simulink model "exemplefir"  (Simulink 7.1)
settings: Solver=FixedStepDiscrete  StartTime=0.0  StopTime=10.0  FixedStep=0.001  RelTol=1e-3
undefined symbols (not defined in the file or in its folder): get, magnitude
libraries: dspbuff3 x2, dspxfrm3 x2, dspsnks4 x2, dspsrcs4 x2, dspsigops x2
settings Model: Creator=Administrateur  LastModifiedBy=Administrateur
settings OptimizationCC: OptimizeModelRefInitCode=on  LifeSpan=1
settings HardwareCC: ProdBitPerInt=16  ProdEndianess=LittleEndian  ProdWordSize=16  ProdHWDeviceType=16-bit Generic
settings RTWCC: SystemTargetFile=dspic.tlc  TemplateMakefile=dspic_pic30_gcc.tmf  PostCodeGenCommand=dsPIC_Compile()  Description=Embedded Target for Microchip dsPIC (real-time)  ProcessScript=dspic_make_rtw_hook
settings CodeAppCC: IgnoreCustomStorageClasses=off
settings STFCustomTargetCC: ModelReferenceCompliant=off  IncludeMdlTerminateFcn=off  CombineOutputUpdateFcns=on  SuppressErrorStatus=on  ERTCustomFileBanners=on  SupportContinuousTime=off  SupportNonInlinedSFcns=off  SystemTargetFile=dspic.tlc
settings ERTTargetCC: ModelReferenceCompliant=off  CompOptLevelCompliant=off  IncludeMdlTerminateFcn=off  SuppressErrorStatus=on  ERTFirstTimeCompliant=off  ModelStepFunctionPrototypeControlCompliant=off  ExtModeMexFile=noextcomm  InlinedParameterPlacement=NonHierarchical  ERTSrcFileBannerTemplate=dsPIC_code_template.cgt  ERTHdrFileBannerTemplate=dsPIC_code_template.cgt  ERTDataSrcFileTemplate=dsPIC_code_template.cgt  ERTDataHdrFileTemplate=dsPIC_code_template.cgt  ERTCustomFileTemplate=dsPIC_main.tlc
settings CustomProperty: DataType=string  Value=C:\PROGRA~1\MATLAB\R2008a\bin\win32\gmake

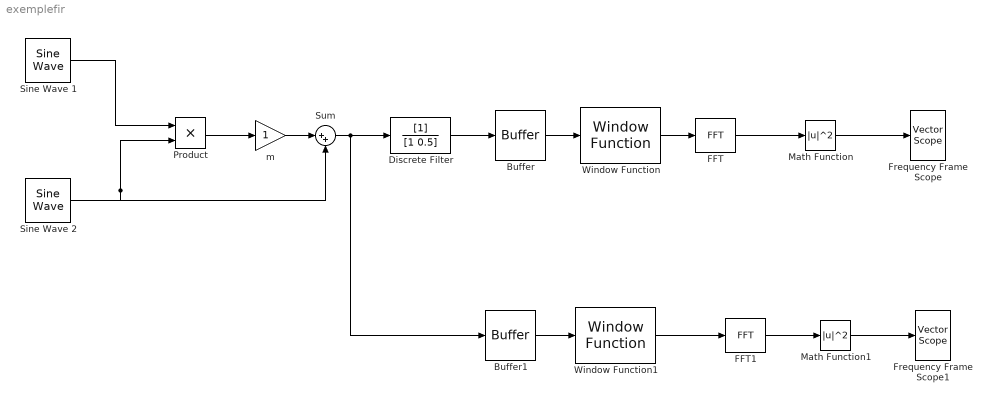
== system exemplefir ==
  Buffer : dspbuff3/Buffer  N=64  V=0  ic=0
  Buffer1 : dspbuff3/Buffer  N=64  V=0  ic=0
  Discrete Filter : DiscreteFilter  Denominator=[1 0.5]  SampleTime=0.1
  FFT : dspxfrm3/FFT  DialogController=dspDDGCreate  DialogControllerArgs=DataTag0  CompMethod=Table lookup  TableOpt=Speed  BitRevOrder=off  InheritFFTLength=on  FFTLength=64  SkipNorm=on  roundingMode=Floor  overflowMode=off
  FFT1 : dspxfrm3/FFT  DialogController=dspDDGCreate  DialogControllerArgs=DataTag1  CompMethod=Table lookup  TableOpt=Speed  BitRevOrder=off  InheritFFTLength=on  FFTLength=64  SkipNorm=on  roundingMode=Floor  overflowMode=off
  Frequency Frame Scope : dspsnks4/Vector Scope  DialogController=dspdialog.VectorScope  DialogControllerArgs=DataTag2  ScopeProperties=on  Domain=Frequency  HorizSpan=1  DisplayProperties=off  AxisGrid=on  Memory=off  FrameNumber=on  AxisLegend=off  AxisZoom=off  OpenScopeAtSimStart=on  OpenScopeImmediately=off  FigPos=get(0,'defaultfigureposition')  AxisProperties=off  XUnits=Hertz  XRange=[0...Fs/2]  InheritXIncr=on  XIncr=1  XLabel=Time  XLimit=Auto  XMin=0  XMax=1  XStart=0  YUnits=dB  YLabel=Amplitude  LineProperties=off
      settings: YMin=-10  YMax=10
  Frequency Frame Scope1 : dspsnks4/Vector Scope  DialogController=dspdialog.VectorScope  DialogControllerArgs=DataTag3  ScopeProperties=on  Domain=Frequency  HorizSpan=1  DisplayProperties=off  AxisGrid=on  Memory=off  FrameNumber=on  AxisLegend=off  AxisZoom=off  OpenScopeAtSimStart=on  OpenScopeImmediately=off  FigPos=get(0,'defaultfigureposition')  AxisProperties=off  XUnits=Hertz  XRange=[0...Fs/2]  InheritXIncr=on  XIncr=1  XLabel=Time  XLimit=Auto  XMin=0  XMax=1  XStart=0  YUnits=dB  YLabel=Amplitude  LineProperties=off
      settings: YMin=-10  YMax=10
  Math Function : Math  Operator=magnitude^2  OutDataType=sfix(16)  OutScaling=2^0  SaturateOnIntegerOverflow=on
  Math Function1 : Math  Operator=magnitude^2  OutDataType=sfix(16)  OutScaling=2^0  SaturateOnIntegerOverflow=on
  Product : Product  OutDataType=sfix(16)  OutScaling=2^0  RndMeth=Zero
  Sine Wave 1 : dspsrcs4/Sine Wave  Amplitude=1  Frequency=100  Phase=0  SampleMode=Discrete  OutComplex=Real  CompMethod=Trigonometric fcn  TableSize=Speed  SampleTime=1/10  SamplesPerFrame=1  dataType=double  wordLen=16  udDataType=sfix(16)  fracBitsMode=Best precision  numFracBits=15  ResetState=Restart at time zero
  Sine Wave 2 : dspsrcs4/Sine Wave  Amplitude=1  Frequency=100  Phase=0  SampleMode=Discrete  OutComplex=Real  CompMethod=Trigonometric fcn  TableSize=Speed  SampleTime=1/10  SamplesPerFrame=1  dataType=double  wordLen=16  udDataType=sfix(16)  fracBitsMode=Best precision  numFracBits=15  ResetState=Restart at time zero
  Sum : Sum  Inputs=|++  OutDataType=sfix(16)  OutScaling=2^0
  Window Function : dspsigops/Window Function  DialogController=dspDDGCreate  DialogControllerArgs=DataTag4  winmode=Apply window to input  wintype=Boxcar  sampmode=Continuous  samptime=1  N=64  Rs=50  beta=10  winsamp=Symmetric  UserWindow=hamming  OptParams=off  UserParams={'symmetric'}  dataType=double  isSigned=on  wordLen=16  udDataType=sfix(16)  fracBitsMode=Best precision  numFracBits=15  roundingMode=Floor  overflowMode=off  numSidelobes=4  sidelobeLevel=-30
  Window Function1 : dspsigops/Window Function  DialogController=dspDDGCreate  DialogControllerArgs=DataTag5  winmode=Apply window to input  wintype=Boxcar  sampmode=Continuous  samptime=1  N=64  Rs=50  beta=10  winsamp=Symmetric  UserWindow=hamming  OptParams=off  UserParams={'symmetric'}  dataType=double  isSigned=on  wordLen=16  udDataType=sfix(16)  fracBitsMode=Best precision  numFracBits=15  roundingMode=Floor  overflowMode=off  numSidelobes=4  sidelobeLevel=-30
  m : Gain  ParameterDataType=sfix(16)  ParameterScaling=2^0  OutDataType=sfix(16)  OutScaling=2^0
  wires:
  Sine Wave 1/1 -> Product/1
  Sine Wave 2/1 -> Product/2, Sum/2
  Product/1 -> m/1
  m/1 -> Sum/1
  Discrete Filter/1 -> Buffer/1
  FFT/1 -> Math Function/1
  Buffer/1 -> Window Function/1
  Window Function/1 -> FFT/1
  Math Function/1 -> Frequency Frame Scope/1
  FFT1/1 -> Math Function1/1
  Buffer1/1 -> Window Function1/1
  Window Function1/1 -> FFT1/1
  Math Function1/1 -> Frequency Frame Scope1/1
  Sum/1 -> Discrete Filter/1, Buffer1/1
